simulink model "ids_sim_harness"  (R2024a)
settings: Solver=FixedStepDiscrete  StartTime=0.0  StopTime=130  FixedStep=0.1  RelTol=1e-3
model workspace (MAT data in the model file):
  A_btnAck = [0 0.1 0.2 0.3 0.4 0.5 0.6 0.7 0.8 0.9 1 1.1 ... (2602 elements, 1301x2)]
  A_btnArm = [0 0.1 0.2 0.3 0.4 0.5 0.6 0.7 0.8 0.9 1 1.1 ... (2602 elements, 1301x2)]
  A_btnSiren = [0 0.1 0.2 0.3 0.4 0.5 0.6 0.7 0.8 0.9 1 1.1 ... (2602 elements, 1301x2)]
  A_gps = [0 0.1 0.2 0.3 0.4 0.5 0.6 0.7 0.8 0.9 1 1.1 ... (5204 elements, 1301x4)]
  A_gyro = [0 0.1 0.2 0.3 0.4 0.5 0.6 0.7 0.8 0.9 1 1.1 ... (5204 elements, 1301x4)]
  A_lux = [0 0.1 0.2 0.3 0.4 0.5 0.6 0.7 0.8 0.9 1 1.1 ... (2602 elements, 1301x2)]
  A_ori = [0 0.1 0.2 0.3 0.4 0.5 0.6 0.7 0.8 0.9 1 1.1 ... (5204 elements, 1301x4)]
  A_role = [0 0.1 0.2 0.3 0.4 0.5 0.6 0.7 0.8 0.9 1 1.1 ... (2602 elements, 1301x2)]
  B_btnAck = [0 0.1 0.2 0.3 0.4 0.5 0.6 0.7 0.8 0.9 1 1.1 ... (2602 elements, 1301x2)]
  B_btnArm = [0 0.1 0.2 0.3 0.4 0.5 0.6 0.7 0.8 0.9 1 1.1 ... (2602 elements, 1301x2)]
  B_btnSiren = [0 0.1 0.2 0.3 0.4 0.5 0.6 0.7 0.8 0.9 1 1.1 ... (2602 elements, 1301x2)]
  B_gps = [0 0.1 0.2 0.3 0.4 0.5 0.6 0.7 0.8 0.9 1 1.1 ... (5204 elements, 1301x4)]
  B_gyro = [0 0.1 0.2 0.3 0.4 0.5 0.6 0.7 0.8 0.9 1 1.1 ... (5204 elements, 1301x4)]
  B_lux = [0 0.1 0.2 0.3 0.4 0.5 0.6 0.7 0.8 0.9 1 1.1 ... (2602 elements, 1301x2)]
  B_ori = [0 0.1 0.2 0.3 0.4 0.5 0.6 0.7 0.8 0.9 1 1.1 ... (5204 elements, 1301x4)]
  B_role = [0 0.1 0.2 0.3 0.4 0.5 0.6 0.7 0.8 0.9 1 1.1 ... (2602 elements, 1301x2)]
(part 2 of 2)

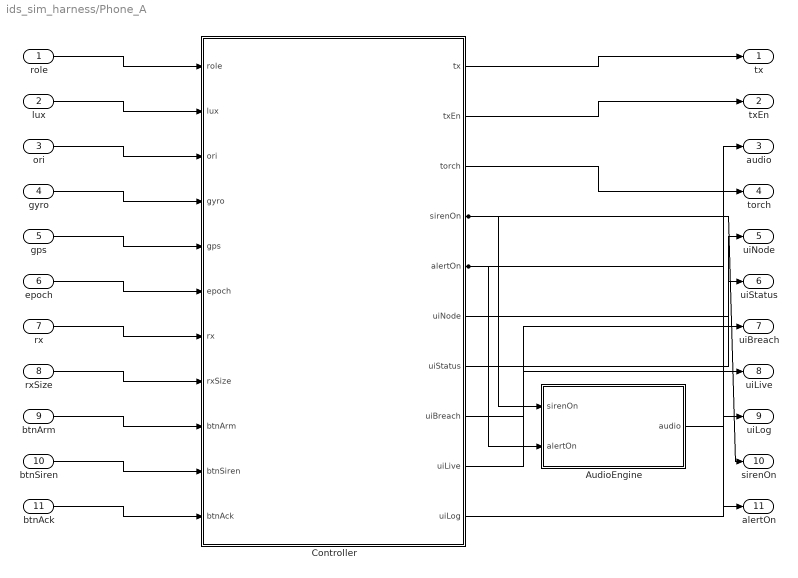
== system ids_sim_harness/Phone_A ==
  role : Inport
  lux : Inport  Port=2
  ori : Inport  Port=3
  gyro : Inport  Port=4
  gps : Inport  Port=5
  epoch : Inport  Port=6
  rx : Inport  Port=7
  rxSize : Inport  Port=8
  btnArm : Inport  Port=9
  btnSiren : Inport  Port=10
  btnAck : Inport  Port=11
  AudioEngine : MATLAB Function  TreatAsAtomicUnit=on
  Controller : MATLAB Function  TreatAsAtomicUnit=on
  tx : Outport
  txEn : Outport  Port=2
  audio : Outport  Port=3
  torch : Outport  Port=4
  uiNode : Outport  Port=5
  uiStatus : Outport  Port=6
  uiBreach : Outport  Port=7
  uiLive : Outport  Port=8
  uiLog : Outport  Port=9
  sirenOn : Outport  Port=10
  alertOn : Outport  Port=11
  wires:
  role/1 -> Controller/1(role)
  lux/1 -> Controller/2(lux)
  ori/1 -> Controller/3(ori)
  gyro/1 -> Controller/4(gyro)
  gps/1 -> Controller/5(gps)
  epoch/1 -> Controller/6(epoch)
  rx/1 -> Controller/7(rx)
  rxSize/1 -> Controller/8(rxSize)
  btnArm/1 -> Controller/9(btnArm)
  btnSiren/1 -> Controller/10(btnSiren)
  btnAck/1 -> Controller/11(btnAck)
  Controller/1(tx) -> tx/1
  Controller/2(txEn) -> txEn/1
  Controller/3(torch) -> torch/1
  Controller/4(sirenOn) -> AudioEngine/1(sirenOn), sirenOn/1
  Controller/5(alertOn) -> AudioEngine/2(alertOn), alertOn/1
  Controller/6(uiNode) -> uiNode/1
  Controller/7(uiStatus) -> uiStatus/1
  Controller/8(uiBreach) -> uiBreach/1
  Controller/9(uiLive) -> uiLive/1
  Controller/10(uiLog) -> uiLog/1
  AudioEngine/1(audio) -> audio/1

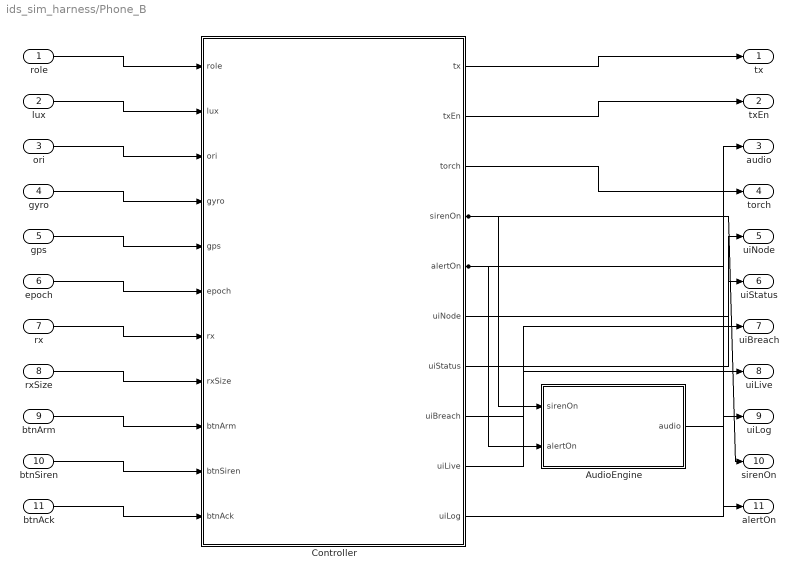
== system ids_sim_harness/Phone_B ==
  role : Inport
  lux : Inport  Port=2
  ori : Inport  Port=3
  gyro : Inport  Port=4
  gps : Inport  Port=5
  epoch : Inport  Port=6
  rx : Inport  Port=7
  rxSize : Inport  Port=8
  btnArm : Inport  Port=9
  btnSiren : Inport  Port=10
  btnAck : Inport  Port=11
  AudioEngine : MATLAB Function  TreatAsAtomicUnit=on
  Controller : MATLAB Function  TreatAsAtomicUnit=on
  tx : Outport
  txEn : Outport  Port=2
  audio : Outport  Port=3
  torch : Outport  Port=4
  uiNode : Outport  Port=5
  uiStatus : Outport  Port=6
  uiBreach : Outport  Port=7
  uiLive : Outport  Port=8
  uiLog : Outport  Port=9
  sirenOn : Outport  Port=10
  alertOn : Outport  Port=11
  wires:
  role/1 -> Controller/1(role)
  lux/1 -> Controller/2(lux)
  ori/1 -> Controller/3(ori)
  gyro/1 -> Controller/4(gyro)
  gps/1 -> Controller/5(gps)
  epoch/1 -> Controller/6(epoch)
  rx/1 -> Controller/7(rx)
  rxSize/1 -> Controller/8(rxSize)
  btnArm/1 -> Controller/9(btnArm)
  btnSiren/1 -> Controller/10(btnSiren)
  btnAck/1 -> Controller/11(btnAck)
  Controller/1(tx) -> tx/1
  Controller/2(txEn) -> txEn/1
  Controller/3(torch) -> torch/1
  Controller/4(sirenOn) -> AudioEngine/1(sirenOn), sirenOn/1
  Controller/5(alertOn) -> AudioEngine/2(alertOn), alertOn/1
  Controller/6(uiNode) -> uiNode/1
  Controller/7(uiStatus) -> uiStatus/1
  Controller/8(uiBreach) -> uiBreach/1
  Controller/9(uiLive) -> uiLive/1
  Controller/10(uiLog) -> uiLog/1
  AudioEngine/1(audio) -> audio/1

== matlab function ids_sim_harness/Phone_A/Controller ==
  data: role input; tx output; lux input; ori input; gyro input; gps input; epoch input; rx input; rxSize input; btnArm input; btnSiren input; btnAck input; txEn output; torch output; sirenOn output; alertOn output; uiNode output; uiStatus output; uiBreach output; uiLive output; uiLog output
function [tx, txEn, torch, sirenOn, alertOn, uiNode, uiStatus, uiBreach, uiLive, uiLog] = controller(role, lux, ori, gyro, gps, epoch, rx, rxSize, btnArm, btnSiren, btnAck)
%#codegen
% Runs the Security Node and the Monitoring Console logic. Only the role
% selected by "role" is active, the other one is held in reset.
% Load the constants once at compile time so they become C literals.
P = coder.const(ids_params());
% "persistent" = a C static variable. Values survive between calls, which
% is how the block remembers its state from one 0.1 s step to the next.
persistent N C
if isempty(N)                     % true only on the very first call
    N = node_init();
    C = console_init(P.logLen);
end
% role comes from the Button: 1 = node, 2 = console. Comparing with 1.5 is
% robust to float or integer typing of the signal.
isNode = double(role(1)) < 1.5;
% Convert Simulink signals to plain doubles for the step functions.
rxd = double(rx(:));
rxs = double(rxSize(1));
t   = double(epoch(1));
% Both state machines run every step. The inactive one gets active = false
% and just resets itself. The transpose (apostrophe) makes row vectors.
[N, txN, enN, torchD, uiNode] = node_step(N, isNode, double(lux(1)), double(ori(:)'), double(gyro(:)'), double(gps(:)'), t, rxd, rxs, P);
[C, txC, enC, uiStatus, uiBreach, uiLive, uiLog] = console_step(C, ~isNode, double(btnArm(1)), double(btnSiren(1)), double(btnAck(1)), t, rxd, rxs, P);
% Pick the packet of the active role.
if isNode
    tx = txN;
    txEn = enN;
else
    tx = txC;
    txEn = enC;
end
% Outputs for the rest of the diagram. The Android ToApp block needs an int32.
torch   = int32(torchD);
sirenOn = double(isNode && N.siren > 0);
alertOn = double(~isNode && C.alert > 0);
end

== matlab function ids_sim_harness/WiFi_Network ==
  data: txA input; rxA output; enA input; txB input; enB input; szA output; rxB output; szB output
function [rxA, szA, rxB, szB] = wifi(txA, enA, txB, enB)
% Delivers each phone's datagrams to the other phone, dropping a fraction.
persistent s
if isempty(s), s = 12345; end
loss = 0.2;
s = mod(1664525*s + 1013904223, 4294967296); uA = s/4294967296;
s = mod(1664525*s + 1013904223, 4294967296); uB = s/4294967296;
rxB = txA; szB = 0;
if enA && uA >= loss, szB = 128; end
rxA = txB; szA = 0;
if enB && uB >= loss, szA = 128; end

== matlab function ids_sim_harness/Phone_A/AudioEngine ==
  data: sirenOn input; audio output; alertOn input
function audio = audio_engine(sirenOn, alertOn)
%#codegen
P = coder.const(ids_params());
persistent A                      % audio state kept between steps
if isempty(A)
    A = audio_init();
end
% coder.load reads alert_message.mat while the code is being generated, so
% the recorded message becomes a constant array inside the app.
S = coder.load('alert_message.mat', 'msg');
[A, audio] = audio_step(A, sirenOn, alertOn, S.msg, P);
end

== matlab function ids_sim_harness/Phone_B/Controller ==
  data: role input; tx output; lux input; ori input; gyro input; gps input; epoch input; rx input; rxSize input; btnArm input; btnSiren input; btnAck input; txEn output; torch output; sirenOn output; alertOn output; uiNode output; uiStatus output; uiBreach output; uiLive output; uiLog output
function [tx, txEn, torch, sirenOn, alertOn, uiNode, uiStatus, uiBreach, uiLive, uiLog] = controller(role, lux, ori, gyro, gps, epoch, rx, rxSize, btnArm, btnSiren, btnAck)
%#codegen
% Runs the Security Node and the Monitoring Console logic. Only the role
% selected by "role" is active, the other one is held in reset.
% Load the constants once at compile time so they become C literals.
P = coder.const(ids_params());
% "persistent" = a C static variable. Values survive between calls, which
% is how the block remembers its state from one 0.1 s step to the next.
persistent N C
if isempty(N)                     % true only on the very first call
    N = node_init();
    C = console_init(P.logLen);
end
% role comes from the Button: 1 = node, 2 = console. Comparing with 1.5 is
% robust to float or integer typing of the signal.
isNode = double(role(1)) < 1.5;
% Convert Simulink signals to plain doubles for the step functions.
rxd = double(rx(:));
rxs = double(rxSize(1));
t   = double(epoch(1));
% Both state machines run every step. The inactive one gets active = false
% and just resets itself. The transpose (apostrophe) makes row vectors.
[N, txN, enN, torchD, uiNode] = node_step(N, isNode, double(lux(1)), double(ori(:)'), double(gyro(:)'), double(gps(:)'), t, rxd, rxs, P);
[C, txC, enC, uiStatus, uiBreach, uiLive, uiLog] = console_step(C, ~isNode, double(btnArm(1)), double(btnSiren(1)), double(btnAck(1)), t, rxd, rxs, P);
% Pick the packet of the active role.
if isNode
    tx = txN;
    txEn = enN;
else
    tx = txC;
    txEn = enC;
end
% Outputs for the rest of the diagram. The Android ToApp block needs an int32.
torch   = int32(torchD);
sirenOn = double(isNode && N.siren > 0);
alertOn = double(~isNode && C.alert > 0);
end

== matlab function ids_sim_harness/Phone_B/AudioEngine ==
  data: sirenOn input; audio output; alertOn input
function audio = audio_engine(sirenOn, alertOn)
%#codegen
P = coder.const(ids_params());
persistent A                      % audio state kept between steps
if isempty(A)
    A = audio_init();
end
% coder.load reads alert_message.mat while the code is being generated, so
% the recorded message becomes a constant array inside the app.
S = coder.load('alert_message.mat', 'msg');
[A, audio] = audio_step(A, sirenOn, alertOn, S.msg, P);
end
